simulink model "adc_zcu111"  (R2018a)
settings: Solver=VariableStepAuto  StartTime=0.0  StopTime=10.0  RelTol=1e-3
libraries: xbsIndex_r4 x50
settings Model: Creator=qwerty40  LastModifiedBy=qwerty40

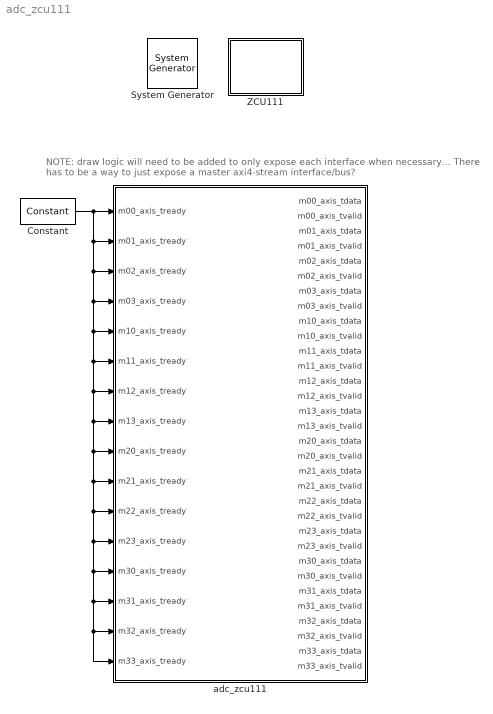
== system adc_zcu111 ==
  note: NOTE: draw logic will need to be added to only expose each interface when necessary...
      | There has to be a way to just expose a master axi4-stream interface/bus?
  " System Generator" : xbsIndex_r4/ System Generator  Tag=genX  xilinxfamily=zynquplusRFSOC  part=xczu28dr  speed=-2-e  package=ffvg1517  synthesis_tool=XST  clock_wrapper=Clock Enables  directory=/home/qwerty40/work_test/mlib_devel/xps_library/xps_models/ADCs/adc_zcu111/sysgen  proj_type=Vivado  Synth_file=Vivado Synthesis Defaults  Impl_file=Vivado Implementation Defaults  testbench=off  simulink_period=1  sysclk_period=10  dcm_input_clock_period=10  incr_netlist=off  trim_vbits=Everywhere in SubSystem  dbl_ovrd=According to Block Masks  core_generation=According to Block Masks  run_coregen=off  deprecated_control=off  eval_field=0  block_type=sysgen
  Constant : xbsIndex_r4/Constant  const=1.0  gui_display_data_type=Boolean  arith_type=Boolean  n_bits=16  bin_pt=14  preci_type=Single  exp_width=8  frac_width=24  explicit_period=off  period=1  equ=P=C  opselect=C  inp2=PCIN>>17  opr=+  inp1=P  carry=CIN  dbl_ovrd=off  block_type=constant
  ZCU111 : Subsystem  Tag=xps:xsg  mask(xsg core config){hw_sys=ZCU111:xczu28dr, clk_src=sys_clk, clk_rate=100, sample_period=1, synthesis_tool=XST}
      mask prompts: hw_sys "Hardware Platform"; clk_src "User IP Clock source"; clk_rate "User IP Clock Rate (MHz)"; sample_period "Sample Period"; synthesis_tool "Synthesis Tool:"
      mask help:
      | The XSG Core Config block is used to configure the System Generator design
      | for the casper_xps toolflow. Settings here are used to configure the
      | Xilinx System Generator block parameters automatically, and control toolflow
      | script  execution. It needs to be at the top level of all designs being compiled
      | with the casper_xps toolflow.
      mask init:
      | xps_xsg_zcu111_conf_mask;
      mask Help: eval('xlWeb([getenv(''MLIB_ROOT''), ''\doc\html\sys_xsg_core_config\sys_xsg_core_config.html''])')
      mask TypeOptions hw_sys: ZCU111:xczu28dr
      mask TypeOptions clk_src: sys_clk | adc_clk
      mask TypeOptions synthesis_tool: Leonardo Spectrum | Synplify | Synplify Pro | XST
      mask Display: fprintf(['ZCU111']);
  adc_zcu111 : Subsystem  Tag=xps:adc_zcu111  mask(adc_zcu111){tile_224_enable_pll=on, tile_224_sample_rate=4096, tile_224_clk_out=256.000, tile_224_ref_clk=512.000, tile_224_axi_stream_clk=0, tile_224_adc_0=on, tile_224_adc0_digital_output=I/Q, tile_224_adc0_dec_mode=2x, tile_224_adc0_sample_per_cycle=8, tile_224_adc0_req_axis_clk=0, tile_224_adc_1=on, tile_224_adc1_digital_output=I/Q, tile_224_adc1_dec_mode=2x, tile_224_adc1_sample_per_cycle=8, tile_224_adc1_req_axis_clk=0, tile_225_enable_pll=on, tile_225_sample_rate=4096, tile_225_clk_out=256.000, tile_225_ref_clk=512.000, tile_225_axi_stream_clk=0, tile_225_adc_0=on, tile_225_adc0_digital_output=I/Q, tile_225_adc0_dec_mode=2x, tile_225_adc0_sample_per_cycle=8, tile_225_adc0_req_axis_clk=0, tile_225_adc_1=on, tile_225_adc1_digital_output=I/Q, tile_225_adc1_dec_mode=2x, tile_225_adc1_sample_per_cycle=8, tile_225_adc1_req_axis_clk=0, tile_226_enable_pll=on, tile_226_sample_rate=4096, tile_226_clk_out=256.000, tile_226_ref_clk=512.000, tile_226_axi_stream_clk=0, tile_226_adc_0=on, tile_226_adc0_digital_output=I/Q, tile_226_adc0_dec_mode=2x, tile_226_adc0_sample_per_cycle=8, tile_226_adc0_req_axis_clk=0, tile_226_adc_1=on, tile_226_adc1_digital_output=I/Q, tile_226_adc1_dec_mode=2x, tile_226_adc1_sample_per_cycle=8, tile_226_adc1_req_axis_clk=0, tile_227_enable_pll=on, tile_227_sample_rate=4096, tile_227_clk_out=256.000, tile_227_ref_clk=512.000, tile_227_axi_stream_clk=0, tile_227_adc_0=on, tile_227_adc0_digital_output=I/Q, tile_227_adc0_dec_mode=2x, tile_227_adc0_sample_per_cycle=8, tile_227_adc0_req_axis_clk=0, tile_227_adc_1=on, tile_227_adc1_digital_output=I/Q, tile_227_adc1_dec_mode=2x, tile_227_adc1_sample_per_cycle=8, tile_227_adc1_req_axis_clk=0}
      mask prompts: tile_224_enable_pll "Enable PLL"; tile_224_sample_rate "Sampling Rate (MSPS)"; tile_224_clk_out "Clock Out (MHz)"; tile_224_ref_clk "Reference Clock (MHz)"; tile_224_axi_stream_clk "AXI4-Stream Clock (MHz)"; tile_224_adc_0 "Enable ADC"; tile_224_adc0_digital_output "Digital Output Data"; tile_224_adc0_dec_mode "Decimation Mode"; tile_224_adc0_sample_per_cycle "Samples per AXI4-Stream Cycle"; tile_224_adc_1 "Enable ADC"; tile_224_adc1_digital_output "Digital Output Data"; tile_224_adc1_dec_mode "Decimation Mode"; tile_224_adc1_sample_per_cycle "Samples per AXI4-Stream Cycle"; tile_225_enable_pll "Enable PLL"; tile_225_sample_rate "Sampling Rate (MSPS)"; tile_225_clk_out "Clock Out (MHz)"; tile_225_ref_clk "Reference Clock (MHz)"; tile_225_axi_stream_clk "AXI4-Stream Clock (MHz)"; tile_225_adc_0 "Enable ADC"; tile_225_adc0_digital_output "Digital Output Data"; tile_225_adc0_dec_mode "Decimation Mode"; tile_225_adc0_sample_per_cycle "Samples per AXI4-Stream Cycle"; tile_225_adc_1 "Enable ADC"; tile_225_adc1_digital_output "Digital Output Data"; tile_225_adc1_dec_mode "Decimation Mode"; tile_225_adc1_sample_per_cycle "Samples per AXI4-Stream Cycle"; tile_226_enable_pll "Enable PLL"; tile_226_sample_rate "Sampling Rate (MSPS)"; tile_226_clk_out "Clock Out (MHz)"; tile_226_ref_clk "Reference Clock (MHz)"; tile_226_axi_stream_clk "AXI4-Stream Clock (MHz)"; tile_226_adc_0 "Enable ADC"; tile_226_adc0_digital_output "Digital Output Data"; tile_226_adc0_dec_mode "Decimation Mode"; tile_226_adc0_sample_per_cycle "Samples per AXI4-Stream Cycle"; tile_226_adc_1 "Enable ADC"; tile_226_adc1_digital_output "Digital Output Data"; tile_226_adc1_dec_mode "Decimation Mode"; tile_226_adc1_sample_per_cycle "Samples per AXI4-Stream Cycle"; tile_227_enable_pll "Enable PLL"; tile_227_sample_rate "Sampling Rate (MSPS)"; tile_227_clk_out "Clock Out (MHz)"; tile_227_ref_clk "Reference Clock (MHz)"; tile_227_axi_stream_clk "AXI4-Stream Clock (MHz)"; tile_227_adc_0 "Enable ADC"; tile_227_adc0_digital_output "Digital Output Data"; tile_227_adc0_dec_mode "Decimation Mode"; tile_227_adc0_sample_per_cycle "Samples per AXI4-Stream Cycle"; tile_227_adc_1 "Enable ADC"; tile_227_adc1_digital_output "Digital Output Data"; tile_227_adc1_dec_mode "Decimation Mode"; tile_227_adc1_sample_per_cycle "Samples per AXI4-Stream Cycle"
      mask init:
      | %adc_zcu111_mask;
      mask Help: eval('xlWeb([getenv(''MLIB_ROOT''), ''\doc\html\adc_zcu111\adc_zcu111.html''])')
      mask TypeOptions tile_224_clk_out: 32.000 | 64.000 | 128.000 | 256.000
      mask TypeOptions tile_224_ref_clk: 103.261 | 104.136 | 105.026 | 105.931 | 106.852 | 107.790 | 108.743 | 109.714 | 110.703 | 111.709 | 112.734 | 113.778 | 114.841 | 115.925 | 117.029 | 118.154 | 119.301 | 120.471 | 121.663 | 122.880 | 124.121 | 125.388 | 126.680 | 128.000 | 129.347 | 130.723 | 132.129 | 133.565 | 135.033 | 136.533 | 138.067 | 139.636 | 141.241 | 142.884 | 144.565 | 146.286 | 148.048 | 149.854 | 151.704 | 153.600 | 155.544 | 157.539 | 159.584 | 161.684 | 163.840 | 166.054 | 168.329 | 170.667 | 173.070 | 175.543 | 178.087 | 180.706 | 183.403 | 186.182 | 189.046 | 192.000 | 195.048 | 198.194 | 201.443 | 204.800 | 208.271 | 211.862 | 215.579 | 219.429 | 223.418 | 227.556 | 231.849 | 236.308 | 240.941 | 245.760 | 250.776 | 256.000 | 261.447 | 267.130 | 273.067 | 279.273 | 285.767 | 292.571 | 299.707 | 307.200 | 315.077 | 323.368 | 332.108 | 341.333 | 351.086 | 361.412 | 372.364 | 384.000 | 396.387 | 409.600 | 423.724 | 438.857 | 455.111 | 472.615 | 491.520 | 512.000 | 534.261 | 558.546 | 585.143 | 614.400 | 646.737 | 682.667 | 722.824 | 768.000
      mask TypeOptions tile_224_adc0_digital_output: I/Q | Real
      mask TypeOptions tile_224_adc0_dec_mode: 1x | 2x | 4x | 8x
      mask TypeOptions tile_224_adc0_sample_per_cycle: 1 | 2 | 3 | 4 | 5 | 6 | 7 | 8
      mask TypeOptions tile_224_adc1_digital_output: I/Q | Real
      mask TypeOptions tile_224_adc1_dec_mode: 1x | 2x | 4x | 8x
      mask TypeOptions tile_224_adc1_sample_per_cycle: 1 | 2 | 3 | 4 | 5 | 6 | 7 | 8
      mask TypeOptions tile_225_clk_out: 32.000 | 64.000 | 128.000 | 256.000
      mask TypeOptions tile_225_ref_clk: 103.261 | 104.136 | 105.026 | 105.931 | 106.852 | 107.790 | 108.743 | 109.714 | 110.703 | 111.709 | 112.734 | 113.778 | 114.841 | 115.925 | 117.029 | 118.154 | 119.301 | 120.471 | 121.663 | 122.880 | 124.121 | 125.388 | 126.680 | 128.000 | 129.347 | 130.723 | 132.129 | 133.565 | 135.033 | 136.533 | 138.067 | 139.636 | 141.241 | 142.884 | 144.565 | 146.286 | 148.048 | 149.854 | 151.704 | 153.600 | 155.544 | 157.539 | 159.584 | 161.684 | 163.840 | 166.054 | 168.329 | 170.667 | 173.070 | 175.543 | 178.087 | 180.706 | 183.403 | 186.182 | 189.046 | 192.000 | 195.048 | 198.194 | 201.443 | 204.800 | 208.271 | 211.862 | 215.579 | 219.429 | 223.418 | 227.556 | 231.849 | 236.308 | 240.941 | 245.760 | 250.776 | 256.000 | 261.447 | 267.130 | 273.067 | 279.273 | 285.767 | 292.571 | 299.707 | 307.200 | 315.077 | 323.368 | 332.108 | 341.333 | 351.086 | 361.412 | 372.364 | 384.000 | 396.387 | 409.600 | 423.724 | 438.857 | 455.111 | 472.615 | 491.520 | 512.000 | 534.261 | 558.546 | 585.143 | 614.400 | 646.737 | 682.667 | 722.824 | 768.000
      mask TypeOptions tile_225_adc0_digital_output: I/Q | Real
      mask TypeOptions tile_225_adc0_dec_mode: 1x | 2x | 4x | 8x
      mask TypeOptions tile_225_adc0_sample_per_cycle: 1 | 2 | 3 | 4 | 5 | 6 | 7 | 8
      mask TypeOptions tile_225_adc1_digital_output: I/Q | Real
      mask TypeOptions tile_225_adc1_dec_mode: 1x | 2x | 4x | 8x
      mask TypeOptions tile_225_adc1_sample_per_cycle: 1 | 2 | 3 | 4 | 5 | 6 | 7 | 8
      mask TypeOptions tile_226_clk_out: 32.000 | 64.000 | 128.000 | 256.000
      mask TypeOptions tile_226_ref_clk: 103.261 | 104.136 | 105.026 | 105.931 | 106.852 | 107.790 | 108.743 | 109.714 | 110.703 | 111.709 | 112.734 | 113.778 | 114.841 | 115.925 | 117.029 | 118.154 | 119.301 | 120.471 | 121.663 | 122.880 | 124.121 | 125.388 | 126.680 | 128.000 | 129.347 | 130.723 | 132.129 | 133.565 | 135.033 | 136.533 | 138.067 | 139.636 | 141.241 | 142.884 | 144.565 | 146.286 | 148.048 | 149.854 | 151.704 | 153.600 | 155.544 | 157.539 | 159.584 | 161.684 | 163.840 | 166.054 | 168.329 | 170.667 | 173.070 | 175.543 | 178.087 | 180.706 | 183.403 | 186.182 | 189.046 | 192.000 | 195.048 | 198.194 | 201.443 | 204.800 | 208.271 | 211.862 | 215.579 | 219.429 | 223.418 | 227.556 | 231.849 | 236.308 | 240.941 | 245.760 | 250.776 | 256.000 | 261.447 | 267.130 | 273.067 | 279.273 | 285.767 | 292.571 | 299.707 | 307.200 | 315.077 | 323.368 | 332.108 | 341.333 | 351.086 | 361.412 | 372.364 | 384.000 | 396.387 | 409.600 | 423.724 | 438.857 | 455.111 | 472.615 | 491.520 | 512.000 | 534.261 | 558.546 | 585.143 | 614.400 | 646.737 | 682.667 | 722.824 | 768.000
      mask TypeOptions tile_226_adc0_digital_output: I/Q | Real
      mask TypeOptions tile_226_adc0_dec_mode: 1x | 2x | 4x | 8x
      mask TypeOptions tile_226_adc0_sample_per_cycle: 1 | 2 | 3 | 4 | 5 | 6 | 7 | 8
      mask TypeOptions tile_226_adc1_digital_output: I/Q | Real
      mask TypeOptions tile_226_adc1_dec_mode: 1x | 2x | 4x | 8x
      mask TypeOptions tile_226_adc1_sample_per_cycle: 1 | 2 | 3 | 4 | 5 | 6 | 7 | 8
      mask TypeOptions tile_227_clk_out: 32.000 | 64.000 | 128.000 | 256.000
      mask TypeOptions tile_227_ref_clk: 103.261 | 104.136 | 105.026 | 105.931 | 106.852 | 107.790 | 108.743 | 109.714 | 110.703 | 111.709 | 112.734 | 113.778 | 114.841 | 115.925 | 117.029 | 118.154 | 119.301 | 120.471 | 121.663 | 122.880 | 124.121 | 125.388 | 126.680 | 128.000 | 129.347 | 130.723 | 132.129 | 133.565 | 135.033 | 136.533 | 138.067 | 139.636 | 141.241 | 142.884 | 144.565 | 146.286 | 148.048 | 149.854 | 151.704 | 153.600 | 155.544 | 157.539 | 159.584 | 161.684 | 163.840 | 166.054 | 168.329 | 170.667 | 173.070 | 175.543 | 178.087 | 180.706 | 183.403 | 186.182 | 189.046 | 192.000 | 195.048 | 198.194 | 201.443 | 204.800 | 208.271 | 211.862 | 215.579 | 219.429 | 223.418 | 227.556 | 231.849 | 236.308 | 240.941 | 245.760 | 250.776 | 256.000 | 261.447 | 267.130 | 273.067 | 279.273 | 285.767 | 292.571 | 299.707 | 307.200 | 315.077 | 323.368 | 332.108 | 341.333 | 351.086 | 361.412 | 372.364 | 384.000 | 396.387 | 409.600 | 423.724 | 438.857 | 455.111 | 472.615 | 491.520 | 512.000 | 534.261 | 558.546 | 585.143 | 614.400 | 646.737 | 682.667 | 722.824 | 768.000
      mask TypeOptions tile_227_adc0_digital_output: I/Q | Real
      mask TypeOptions tile_227_adc0_dec_mode: 1x | 2x | 4x | 8x
      mask TypeOptions tile_227_adc0_sample_per_cycle: 1 | 2 | 3 | 4 | 5 | 6 | 7 | 8
      mask TypeOptions tile_227_adc1_digital_output: I/Q | Real
      mask TypeOptions tile_227_adc1_dec_mode: 1x | 2x | 4x | 8x
      mask TypeOptions tile_227_adc1_sample_per_cycle: 1 | 2 | 3 | 4 | 5 | 6 | 7 | 8
      mask DialogControl adc_tile_224 Prompt: ADC Tile 224
      mask DialogControl pll_clocking_config_224 Prompt: PLL and Clocking Configuration
      mask DialogControl tile_224_adc0 Prompt: ADC 0
      mask DialogControl tile_224_adc0_data_settings Prompt: Data Settings
      mask DialogControl tile_224_adc0_req_axis_clk_label Prompt: Required AXI4-Stream clock:
      mask DialogControl tile_224_adc1 Prompt: ADC 1
      mask DialogControl tile_224_adc1_data_settings Prompt: Data Settings
      mask DialogControl tile_224_adc1_req_axis_clk_label Prompt: Required AXI4-Stream clock:
      mask DialogControl adc_tile_225 Prompt: ADC Tile 225
      mask DialogControl pll_clocking_config_225 Prompt: PLL and Clocking Configuration
      mask DialogControl tile_225_adc0 Prompt: ADC 0
      mask DialogControl tile_225_adc0_data_settings Prompt: Data Settings
      mask DialogControl tile_225_adc0_req_axis_clk_label Prompt: Required AXI4-Stream clock:
      mask DialogControl tile_225_adc1 Prompt: ADC 1
      mask DialogControl tile_225_adc1_data_settings Prompt: Data Settings
      mask DialogControl tile_225_adc1_req_axis_clk_label Prompt: Required AXI4-Stream clock:
      mask DialogControl adc_tile_226 Prompt: ADC Tile 226
      mask DialogControl pll_clocking_config_226 Prompt: PLL and Clocking Configuration
      mask DialogControl tile_226_adc0 Prompt: ADC 0
      mask DialogControl tile_226_adc0_data_settings Prompt: Data Settings
      mask DialogControl tile_226_adc0_req_axis_clk_label Prompt: Required AXI4-Stream clock:
      mask DialogControl tile_226_adc1 Prompt: ADC 1
      mask DialogControl tile_226_adc1_data_settings Prompt: Data Settings
      mask DialogControl tile_226_adc1_req_axis_clk_label Prompt: Required AXI4-Stream clock:
      mask DialogControl adc_tile_227 Prompt: ADC Tile 227
      mask DialogControl pll_clocking_config_227 Prompt: PLL and Clocking Configuration
      mask DialogControl tile_227_adc0 Prompt: ADC 0
      mask DialogControl tile_227_adc0_data_settings Prompt: Data Settings
      mask DialogControl tile_227_adc0_req_axis_clk_label Prompt: Required AXI4-Stream clock:
      mask DialogControl tile_227_adc1 Prompt: ADC 1
      mask DialogControl tile_227_adc1_data_settings Prompt: Data Settings
      mask DialogControl tile_227_adc1_req_axis_clk_label Prompt: Required AXI4-Stream clock:
  wires:
  Constant/1 -> adc_zcu111/4(m03_axis_tready), adc_zcu111/5(m10_axis_tready), adc_zcu111/6(m11_axis_tready), adc_zcu111/7(m12_axis_tready), adc_zcu111/8(m13_axis_tready), adc_zcu111/9(m20_axis_tready), adc_zcu111/10(m21_axis_tready), adc_zcu111/11(m22_axis_tready), adc_zcu111/13(m30_axis_tready), adc_zcu111/14(m31_axis_tready), adc_zcu111/15(m32_axis_tready), adc_zcu111/16(m33_axis_tready), adc_zcu111/12(m23_axis_tready), adc_zcu111/3(m02_axis_tready), adc_zcu111/2(m01_axis_tready), adc_zcu111/1(m00_axis_tready)

== system adc_zcu111/ZCU111 ==

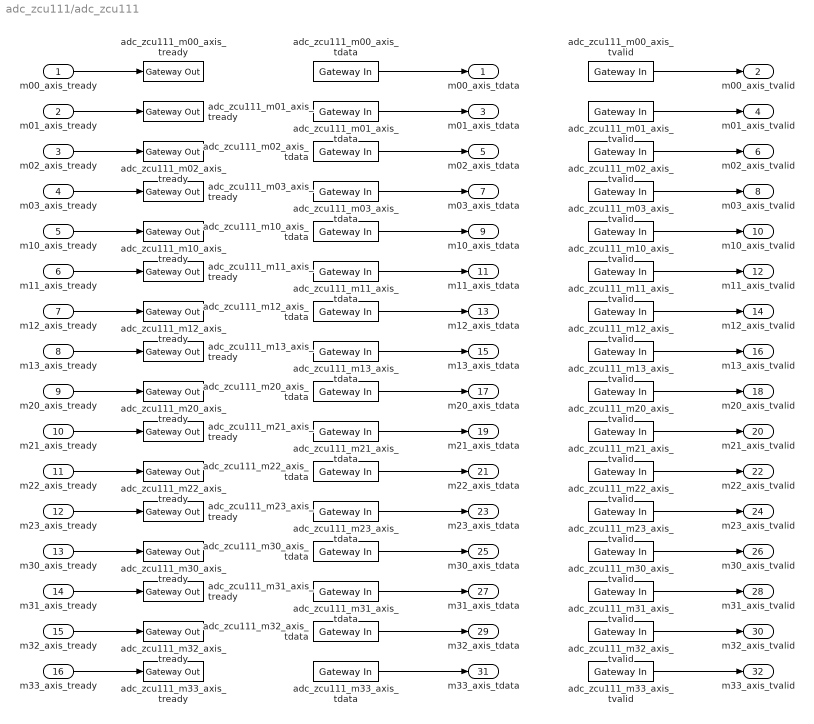
== system adc_zcu111/adc_zcu111 ==
  m00_axis_tready : Inport  OutDataTypeStr=boolean
  m01_axis_tready : Inport  Port=2  OutDataTypeStr=boolean
  m02_axis_tready : Inport  Port=3  OutDataTypeStr=boolean
  m03_axis_tready : Inport  Port=4  OutDataTypeStr=boolean
  m10_axis_tready : Inport  Port=5  OutDataTypeStr=boolean
  m11_axis_tready : Inport  Port=6  OutDataTypeStr=boolean
  m12_axis_tready : Inport  Port=7  OutDataTypeStr=boolean
  m13_axis_tready : Inport  Port=8  OutDataTypeStr=boolean
  m20_axis_tready : Inport  Port=9  OutDataTypeStr=boolean
  m21_axis_tready : Inport  Port=10  OutDataTypeStr=boolean
  m22_axis_tready : Inport  Port=11  OutDataTypeStr=boolean
  m23_axis_tready : Inport  Port=12  OutDataTypeStr=boolean
  m30_axis_tready : Inport  Port=13  OutDataTypeStr=boolean
  m31_axis_tready : Inport  Port=14  OutDataTypeStr=boolean
  m32_axis_tready : Inport  Port=15  OutDataTypeStr=boolean
  m33_axis_tready : Inport  Port=16  OutDataTypeStr=boolean
  adc_zcu111_m00_axis_tdata : xbsIndex_r4/Gateway In  gui_display_data_type=Fixed-point  arith_type="Signed  (2's comp)"  n_bits=128  bin_pt=126  preci_type=Double  exp_width=8  frac_width=24  rows=1  columns=1  quantization="Round  (unbiased: +/- Inf)"  overflow=Saturate  period=1  UseAsADC=off  ADCChannel='1'  interface=None  automatic_assignment=on  address_offset=hex2dec('00')  intf_name=''  intf_description=''  default_value=0  timing_constraint=None  locs_specified=off  LOCs={}  io_standard={}  inherit_from_input=off  hdl_port=on  dbl_ovrd=off  block_type=gatewayin
  adc_zcu111_m00_axis_tready : xbsIndex_r4/Gateway Out  inherit_from_input=on  hdl_port=on  rows=1  columns=1  UseAsDAC=off  DACChannel='1'  interface=None  automatic_assignment=on  address_offset=hex2dec('00')  intf_name=''  intf_description=''  timing_constraint=None  locs_specified=off  LOCs={}  io_standard={}  block_type=gatewayout
  adc_zcu111_m00_axis_tvalid : xbsIndex_r4/Gateway In  gui_display_data_type=Boolean  arith_type=Boolean  n_bits=128  bin_pt=126  preci_type=Double  exp_width=8  frac_width=24  rows=1  columns=1  quantization="Round  (unbiased: +/- Inf)"  overflow=Saturate  period=1  UseAsADC=off  ADCChannel='1'  interface=None  automatic_assignment=on  address_offset=hex2dec('00')  intf_name=''  intf_description=''  default_value=0  timing_constraint=None  locs_specified=off  LOCs={}  io_standard={}  inherit_from_input=off  hdl_port=on  dbl_ovrd=off  block_type=gatewayin
  adc_zcu111_m01_axis_tdata : xbsIndex_r4/Gateway In  gui_display_data_type=Fixed-point  arith_type="Signed  (2's comp)"  n_bits=128  bin_pt=126  preci_type=Double  exp_width=8  frac_width=24  rows=1  columns=1  quantization="Round  (unbiased: +/- Inf)"  overflow=Saturate  period=1  UseAsADC=off  ADCChannel='1'  interface=None  automatic_assignment=on  address_offset=hex2dec('00')  intf_name=''  intf_description=''  default_value=0  timing_constraint=None  locs_specified=off  LOCs={}  io_standard={}  inherit_from_input=off  hdl_port=on  dbl_ovrd=off  block_type=gatewayin
  adc_zcu111_m01_axis_tready : xbsIndex_r4/Gateway Out  inherit_from_input=on  hdl_port=on  rows=1  columns=1  UseAsDAC=off  DACChannel='1'  interface=None  automatic_assignment=on  address_offset=hex2dec('00')  intf_name=''  intf_description=''  timing_constraint=None  locs_specified=off  LOCs={}  io_standard={}  block_type=gatewayout
  adc_zcu111_m01_axis_tvalid : xbsIndex_r4/Gateway In  gui_display_data_type=Boolean  arith_type=Boolean  n_bits=128  bin_pt=126  preci_type=Double  exp_width=8  frac_width=24  rows=1  columns=1  quantization="Round  (unbiased: +/- Inf)"  overflow=Saturate  period=1  UseAsADC=off  ADCChannel='1'  interface=None  automatic_assignment=on  address_offset=hex2dec('00')  intf_name=''  intf_description=''  default_value=0  timing_constraint=None  locs_specified=off  LOCs={}  io_standard={}  inherit_from_input=off  hdl_port=on  dbl_ovrd=off  block_type=gatewayin
  adc_zcu111_m02_axis_tdata : xbsIndex_r4/Gateway In  gui_display_data_type=Fixed-point  arith_type="Signed  (2's comp)"  n_bits=128  bin_pt=126  preci_type=Double  exp_width=8  frac_width=24  rows=1  columns=1  quantization="Round  (unbiased: +/- Inf)"  overflow=Saturate  period=1  UseAsADC=off  ADCChannel='1'  interface=None  automatic_assignment=on  address_offset=hex2dec('00')  intf_name=''  intf_description=''  default_value=0  timing_constraint=None  locs_specified=off  LOCs={}  io_standard={}  inherit_from_input=off  hdl_port=on  dbl_ovrd=off  block_type=gatewayin
  adc_zcu111_m02_axis_tready : xbsIndex_r4/Gateway Out  inherit_from_input=on  hdl_port=on  rows=1  columns=1  UseAsDAC=off  DACChannel='1'  interface=None  automatic_assignment=on  address_offset=hex2dec('00')  intf_name=''  intf_description=''  timing_constraint=None  locs_specified=off  LOCs={}  io_standard={}  block_type=gatewayout
  adc_zcu111_m02_axis_tvalid : xbsIndex_r4/Gateway In  gui_display_data_type=Boolean  arith_type=Boolean  n_bits=128  bin_pt=126  preci_type=Double  exp_width=8  frac_width=24  rows=1  columns=1  quantization="Round  (unbiased: +/- Inf)"  overflow=Saturate  period=1  UseAsADC=off  ADCChannel='1'  interface=None  automatic_assignment=on  address_offset=hex2dec('00')  intf_name=''  intf_description=''  default_value=0  timing_constraint=None  locs_specified=off  LOCs={}  io_standard={}  inherit_from_input=off  hdl_port=on  dbl_ovrd=off  block_type=gatewayin
  adc_zcu111_m03_axis_tdata : xbsIndex_r4/Gateway In  gui_display_data_type=Fixed-point  arith_type="Signed  (2's comp)"  n_bits=128  bin_pt=126  preci_type=Double  exp_width=8  frac_width=24  rows=1  columns=1  quantization="Round  (unbiased: +/- Inf)"  overflow=Saturate  period=1  UseAsADC=off  ADCChannel='1'  interface=None  automatic_assignment=on  address_offset=hex2dec('00')  intf_name=''  intf_description=''  default_value=0  timing_constraint=None  locs_specified=off  LOCs={}  io_standard={}  inherit_from_input=off  hdl_port=on  dbl_ovrd=off  block_type=gatewayin
  adc_zcu111_m03_axis_tready : xbsIndex_r4/Gateway Out  inherit_from_input=on  hdl_port=on  rows=1  columns=1  UseAsDAC=off  DACChannel='1'  interface=None  automatic_assignment=on  address_offset=hex2dec('00')  intf_name=''  intf_description=''  timing_constraint=None  locs_specified=off  LOCs={}  io_standard={}  block_type=gatewayout
  adc_zcu111_m03_axis_tvalid : xbsIndex_r4/Gateway In  gui_display_data_type=Boolean  arith_type=Boolean  n_bits=128  bin_pt=126  preci_type=Double  exp_width=8  frac_width=24  rows=1  columns=1  quantization="Round  (unbiased: +/- Inf)"  overflow=Saturate  period=1  UseAsADC=off  ADCChannel='1'  interface=None  automatic_assignment=on  address_offset=hex2dec('00')  intf_name=''  intf_description=''  default_value=0  timing_constraint=None  locs_specified=off  LOCs={}  io_standard={}  inherit_from_input=off  hdl_port=on  dbl_ovrd=off  block_type=gatewayin
  adc_zcu111_m10_axis_tdata : xbsIndex_r4/Gateway In  gui_display_data_type=Fixed-point  arith_type="Signed  (2's comp)"  n_bits=128  bin_pt=126  preci_type=Double  exp_width=8  frac_width=24  rows=1  columns=1  quantization="Round  (unbiased: +/- Inf)"  overflow=Saturate  period=1  UseAsADC=off  ADCChannel='1'  interface=None  automatic_assignment=on  address_offset=hex2dec('00')  intf_name=''  intf_description=''  default_value=0  timing_constraint=None  locs_specified=off  LOCs={}  io_standard={}  inherit_from_input=off  hdl_port=on  dbl_ovrd=off  block_type=gatewayin
  adc_zcu111_m10_axis_tready : xbsIndex_r4/Gateway Out  inherit_from_input=on  hdl_port=on  rows=1  columns=1  UseAsDAC=off  DACChannel='1'  interface=None  automatic_assignment=on  address_offset=hex2dec('00')  intf_name=''  intf_description=''  timing_constraint=None  locs_specified=off  LOCs={}  io_standard={}  block_type=gatewayout
  adc_zcu111_m10_axis_tvalid : xbsIndex_r4/Gateway In  gui_display_data_type=Boolean  arith_type=Boolean  n_bits=128  bin_pt=126  preci_type=Double  exp_width=8  frac_width=24  rows=1  columns=1  quantization="Round  (unbiased: +/- Inf)"  overflow=Saturate  period=1  UseAsADC=off  ADCChannel='1'  interface=None  automatic_assignment=on  address_offset=hex2dec('00')  intf_name=''  intf_description=''  default_value=0  timing_constraint=None  locs_specified=off  LOCs={}  io_standard={}  inherit_from_input=off  hdl_port=on  dbl_ovrd=off  block_type=gatewayin
  adc_zcu111_m11_axis_tdata : xbsIndex_r4/Gateway In  gui_display_data_type=Fixed-point  arith_type="Signed  (2's comp)"  n_bits=128  bin_pt=126  preci_type=Double  exp_width=8  frac_width=24  rows=1  columns=1  quantization="Round  (unbiased: +/- Inf)"  overflow=Saturate  period=1  UseAsADC=off  ADCChannel='1'  interface=None  automatic_assignment=on  address_offset=hex2dec('00')  intf_name=''  intf_description=''  default_value=0  timing_constraint=None  locs_specified=off  LOCs={}  io_standard={}  inherit_from_input=off  hdl_port=on  dbl_ovrd=off  block_type=gatewayin
  adc_zcu111_m11_axis_tready : xbsIndex_r4/Gateway Out  inherit_from_input=on  hdl_port=on  rows=1  columns=1  UseAsDAC=off  DACChannel='1'  interface=None  automatic_assignment=on  address_offset=hex2dec('00')  intf_name=''  intf_description=''  timing_constraint=None  locs_specified=off  LOCs={}  io_standard={}  block_type=gatewayout
  adc_zcu111_m11_axis_tvalid : xbsIndex_r4/Gateway In  gui_display_data_type=Boolean  arith_type=Boolean  n_bits=128  bin_pt=126  preci_type=Double  exp_width=8  frac_width=24  rows=1  columns=1  quantization="Round  (unbiased: +/- Inf)"  overflow=Saturate  period=1  UseAsADC=off  ADCChannel='1'  interface=None  automatic_assignment=on  address_offset=hex2dec('00')  intf_name=''  intf_description=''  default_value=0  timing_constraint=None  locs_specified=off  LOCs={}  io_standard={}  inherit_from_input=off  hdl_port=on  dbl_ovrd=off  block_type=gatewayin
  adc_zcu111_m12_axis_tdata : xbsIndex_r4/Gateway In  gui_display_data_type=Fixed-point  arith_type="Signed  (2's comp)"  n_bits=128  bin_pt=126  preci_type=Double  exp_width=8  frac_width=24  rows=1  columns=1  quantization="Round  (unbiased: +/- Inf)"  overflow=Saturate  period=1  UseAsADC=off  ADCChannel='1'  interface=None  automatic_assignment=on  address_offset=hex2dec('00')  intf_name=''  intf_description=''  default_value=0  timing_constraint=None  locs_specified=off  LOCs={}  io_standard={}  inherit_from_input=off  hdl_port=on  dbl_ovrd=off  block_type=gatewayin
  adc_zcu111_m12_axis_tready : xbsIndex_r4/Gateway Out  inherit_from_input=on  hdl_port=on  rows=1  columns=1  UseAsDAC=off  DACChannel='1'  interface=None  automatic_assignment=on  address_offset=hex2dec('00')  intf_name=''  intf_description=''  timing_constraint=None  locs_specified=off  LOCs={}  io_standard={}  block_type=gatewayout
  adc_zcu111_m12_axis_tvalid : xbsIndex_r4/Gateway In  gui_display_data_type=Boolean  arith_type=Boolean  n_bits=128  bin_pt=126  preci_type=Double  exp_width=8  frac_width=24  rows=1  columns=1  quantization="Round  (unbiased: +/- Inf)"  overflow=Saturate  period=1  UseAsADC=off  ADCChannel='1'  interface=None  automatic_assignment=on  address_offset=hex2dec('00')  intf_name=''  intf_description=''  default_value=0  timing_constraint=None  locs_specified=off  LOCs={}  io_standard={}  inherit_from_input=off  hdl_port=on  dbl_ovrd=off  block_type=gatewayin
  adc_zcu111_m13_axis_tdata : xbsIndex_r4/Gateway In  gui_display_data_type=Fixed-point  arith_type="Signed  (2's comp)"  n_bits=128  bin_pt=126  preci_type=Double  exp_width=8  frac_width=24  rows=1  columns=1  quantization="Round  (unbiased: +/- Inf)"  overflow=Saturate  period=1  UseAsADC=off  ADCChannel='1'  interface=None  automatic_assignment=on  address_offset=hex2dec('00')  intf_name=''  intf_description=''  default_value=0  timing_constraint=None  locs_specified=off  LOCs={}  io_standard={}  inherit_from_input=off  hdl_port=on  dbl_ovrd=off  block_type=gatewayin
  adc_zcu111_m13_axis_tready : xbsIndex_r4/Gateway Out  inherit_from_input=on  hdl_port=on  rows=1  columns=1  UseAsDAC=off  DACChannel='1'  interface=None  automatic_assignment=on  address_offset=hex2dec('00')  intf_name=''  intf_description=''  timing_constraint=None  locs_specified=off  LOCs={}  io_standard={}  block_type=gatewayout
  adc_zcu111_m13_axis_tvalid : xbsIndex_r4/Gateway In  gui_display_data_type=Boolean  arith_type=Boolean  n_bits=128  bin_pt=126  preci_type=Double  exp_width=8  frac_width=24  rows=1  columns=1  quantization="Round  (unbiased: +/- Inf)"  overflow=Saturate  period=1  UseAsADC=off  ADCChannel='1'  interface=None  automatic_assignment=on  address_offset=hex2dec('00')  intf_name=''  intf_description=''  default_value=0  timing_constraint=None  locs_specified=off  LOCs={}  io_standard={}  inherit_from_input=off  hdl_port=on  dbl_ovrd=off  block_type=gatewayin
  adc_zcu111_m20_axis_tdata : xbsIndex_r4/Gateway In  gui_display_data_type=Fixed-point  arith_type="Signed  (2's comp)"  n_bits=128  bin_pt=126  preci_type=Double  exp_width=8  frac_width=24  rows=1  columns=1  quantization="Round  (unbiased: +/- Inf)"  overflow=Saturate  period=1  UseAsADC=off  ADCChannel='1'  interface=None  automatic_assignment=on  address_offset=hex2dec('00')  intf_name=''  intf_description=''  default_value=0  timing_constraint=None  locs_specified=off  LOCs={}  io_standard={}  inherit_from_input=off  hdl_port=on  dbl_ovrd=off  block_type=gatewayin
  adc_zcu111_m20_axis_tready : xbsIndex_r4/Gateway Out  inherit_from_input=on  hdl_port=on  rows=1  columns=1  UseAsDAC=off  DACChannel='1'  interface=None  automatic_assignment=on  address_offset=hex2dec('00')  intf_name=''  intf_description=''  timing_constraint=None  locs_specified=off  LOCs={}  io_standard={}  block_type=gatewayout
  adc_zcu111_m20_axis_tvalid : xbsIndex_r4/Gateway In  gui_display_data_type=Boolean  arith_type=Boolean  n_bits=128  bin_pt=126  preci_type=Double  exp_width=8  frac_width=24  rows=1  columns=1  quantization="Round  (unbiased: +/- Inf)"  overflow=Saturate  period=1  UseAsADC=off  ADCChannel='1'  interface=None  automatic_assignment=on  address_offset=hex2dec('00')  intf_name=''  intf_description=''  default_value=0  timing_constraint=None  locs_specified=off  LOCs={}  io_standard={}  inherit_from_input=off  hdl_port=on  dbl_ovrd=off  block_type=gatewayin
  adc_zcu111_m21_axis_tdata : xbsIndex_r4/Gateway In  gui_display_data_type=Fixed-point  arith_type="Signed  (2's comp)"  n_bits=128  bin_pt=126  preci_type=Double  exp_width=8  frac_width=24  rows=1  columns=1  quantization="Round  (unbiased: +/- Inf)"  overflow=Saturate  period=1  UseAsADC=off  ADCChannel='1'  interface=None  automatic_assignment=on  address_offset=hex2dec('00')  intf_name=''  intf_description=''  default_value=0  timing_constraint=None  locs_specified=off  LOCs={}  io_standard={}  inherit_from_input=off  hdl_port=on  dbl_ovrd=off  block_type=gatewayin
  adc_zcu111_m21_axis_tready : xbsIndex_r4/Gateway Out  inherit_from_input=on  hdl_port=on  rows=1  columns=1  UseAsDAC=off  DACChannel='1'  interface=None  automatic_assignment=on  address_offset=hex2dec('00')  intf_name=''  intf_description=''  timing_constraint=None  locs_specified=off  LOCs={}  io_standard={}  block_type=gatewayout
  adc_zcu111_m21_axis_tvalid : xbsIndex_r4/Gateway In  gui_display_data_type=Boolean  arith_type=Boolean  n_bits=128  bin_pt=126  preci_type=Double  exp_width=8  frac_width=24  rows=1  columns=1  quantization="Round  (unbiased: +/- Inf)"  overflow=Saturate  period=1  UseAsADC=off  ADCChannel='1'  interface=None  automatic_assignment=on  address_offset=hex2dec('00')  intf_name=''  intf_description=''  default_value=0  timing_constraint=None  locs_specified=off  LOCs={}  io_standard={}  inherit_from_input=off  hdl_port=on  dbl_ovrd=off  block_type=gatewayin
  adc_zcu111_m22_axis_tdata : xbsIndex_r4/Gateway In  gui_display_data_type=Fixed-point  arith_type="Signed  (2's comp)"  n_bits=128  bin_pt=126  preci_type=Double  exp_width=8  frac_width=24  rows=1  columns=1  quantization="Round  (unbiased: +/- Inf)"  overflow=Saturate  period=1  UseAsADC=off  ADCChannel='1'  interface=None  automatic_assignment=on  address_offset=hex2dec('00')  intf_name=''  intf_description=''  default_value=0  timing_constraint=None  locs_specified=off  LOCs={}  io_standard={}  inherit_from_input=off  hdl_port=on  dbl_ovrd=off  block_type=gatewayin
  adc_zcu111_m22_axis_tready : xbsIndex_r4/Gateway Out  inherit_from_input=on  hdl_port=on  rows=1  columns=1  UseAsDAC=off  DACChannel='1'  interface=None  automatic_assignment=on  address_offset=hex2dec('00')  intf_name=''  intf_description=''  timing_constraint=None  locs_specified=off  LOCs={}  io_standard={}  block_type=gatewayout
  adc_zcu111_m22_axis_tvalid : xbsIndex_r4/Gateway In  gui_display_data_type=Boolean  arith_type=Boolean  n_bits=128  bin_pt=126  preci_type=Double  exp_width=8  frac_width=24  rows=1  columns=1  quantization="Round  (unbiased: +/- Inf)"  overflow=Saturate  period=1  UseAsADC=off  ADCChannel='1'  interface=None  automatic_assignment=on  address_offset=hex2dec('00')  intf_name=''  intf_description=''  default_value=0  timing_constraint=None  locs_specified=off  LOCs={}  io_standard={}  inherit_from_input=off  hdl_port=on  dbl_ovrd=off  block_type=gatewayin
  adc_zcu111_m23_axis_tdata : xbsIndex_r4/Gateway In  gui_display_data_type=Fixed-point  arith_type="Signed  (2's comp)"  n_bits=128  bin_pt=126  preci_type=Double  exp_width=8  frac_width=24  rows=1  columns=1  quantization="Round  (unbiased: +/- Inf)"  overflow=Saturate  period=1  UseAsADC=off  ADCChannel='1'  interface=None  automatic_assignment=on  address_offset=hex2dec('00')  intf_name=''  intf_description=''  default_value=0  timing_constraint=None  locs_specified=off  LOCs={}  io_standard={}  inherit_from_input=off  hdl_port=on  dbl_ovrd=off  block_type=gatewayin
  adc_zcu111_m23_axis_tready : xbsIndex_r4/Gateway Out  inherit_from_input=on  hdl_port=on  rows=1  columns=1  UseAsDAC=off  DACChannel='1'  interface=None  automatic_assignment=on  address_offset=hex2dec('00')  intf_name=''  intf_description=''  timing_constraint=None  locs_specified=off  LOCs={}  io_standard={}  block_type=gatewayout
  adc_zcu111_m23_axis_tvalid : xbsIndex_r4/Gateway In  gui_display_data_type=Boolean  arith_type=Boolean  n_bits=128  bin_pt=126  preci_type=Double  exp_width=8  frac_width=24  rows=1  columns=1  quantization="Round  (unbiased: +/- Inf)"  overflow=Saturate  period=1  UseAsADC=off  ADCChannel='1'  interface=None  automatic_assignment=on  address_offset=hex2dec('00')  intf_name=''  intf_description=''  default_value=0  timing_constraint=None  locs_specified=off  LOCs={}  io_standard={}  inherit_from_input=off  hdl_port=on  dbl_ovrd=off  block_type=gatewayin
  adc_zcu111_m30_axis_tdata : xbsIndex_r4/Gateway In  gui_display_data_type=Fixed-point  arith_type="Signed  (2's comp)"  n_bits=128  bin_pt=126  preci_type=Double  exp_width=8  frac_width=24  rows=1  columns=1  quantization="Round  (unbiased: +/- Inf)"  overflow=Saturate  period=1  UseAsADC=off  ADCChannel='1'  interface=None  automatic_assignment=on  address_offset=hex2dec('00')  intf_name=''  intf_description=''  default_value=0  timing_constraint=None  locs_specified=off  LOCs={}  io_standard={}  inherit_from_input=off  hdl_port=on  dbl_ovrd=off  block_type=gatewayin
  adc_zcu111_m30_axis_tready : xbsIndex_r4/Gateway Out  inherit_from_input=on  hdl_port=on  rows=1  columns=1  UseAsDAC=off  DACChannel='1'  interface=None  automatic_assignment=on  address_offset=hex2dec('00')  intf_name=''  intf_description=''  timing_constraint=None  locs_specified=off  LOCs={}  io_standard={}  block_type=gatewayout
  adc_zcu111_m30_axis_tvalid : xbsIndex_r4/Gateway In  gui_display_data_type=Boolean  arith_type=Boolean  n_bits=128  bin_pt=126  preci_type=Double  exp_width=8  frac_width=24  rows=1  columns=1  quantization="Round  (unbiased: +/- Inf)"  overflow=Saturate  period=1  UseAsADC=off  ADCChannel='1'  interface=None  automatic_assignment=on  address_offset=hex2dec('00')  intf_name=''  intf_description=''  default_value=0  timing_constraint=None  locs_specified=off  LOCs={}  io_standard={}  inherit_from_input=off  hdl_port=on  dbl_ovrd=off  block_type=gatewayin
  adc_zcu111_m31_axis_tdata : xbsIndex_r4/Gateway In  gui_display_data_type=Fixed-point  arith_type="Signed  (2's comp)"  n_bits=128  bin_pt=126  preci_type=Double  exp_width=8  frac_width=24  rows=1  columns=1  quantization="Round  (unbiased: +/- Inf)"  overflow=Saturate  period=1  UseAsADC=off  ADCChannel='1'  interface=None  automatic_assignment=on  address_offset=hex2dec('00')  intf_name=''  intf_description=''  default_value=0  timing_constraint=None  locs_specified=off  LOCs={}  io_standard={}  inherit_from_input=off  hdl_port=on  dbl_ovrd=off  block_type=gatewayin
  adc_zcu111_m31_axis_tready : xbsIndex_r4/Gateway Out  inherit_from_input=on  hdl_port=on  rows=1  columns=1  UseAsDAC=off  DACChannel='1'  interface=None  automatic_assignment=on  address_offset=hex2dec('00')  intf_name=''  intf_description=''  timing_constraint=None  locs_specified=off  LOCs={}  io_standard={}  block_type=gatewayout
  adc_zcu111_m31_axis_tvalid : xbsIndex_r4/Gateway In  gui_display_data_type=Boolean  arith_type=Boolean  n_bits=128  bin_pt=126  preci_type=Double  exp_width=8  frac_width=24  rows=1  columns=1  quantization="Round  (unbiased: +/- Inf)"  overflow=Saturate  period=1  UseAsADC=off  ADCChannel='1'  interface=None  automatic_assignment=on  address_offset=hex2dec('00')  intf_name=''  intf_description=''  default_value=0  timing_constraint=None  locs_specified=off  LOCs={}  io_standard={}  inherit_from_input=off  hdl_port=on  dbl_ovrd=off  block_type=gatewayin
  adc_zcu111_m32_axis_tdata : xbsIndex_r4/Gateway In  gui_display_data_type=Fixed-point  arith_type="Signed  (2's comp)"  n_bits=128  bin_pt=126  preci_type=Double  exp_width=8  frac_width=24  rows=1  columns=1  quantization="Round  (unbiased: +/- Inf)"  overflow=Saturate  period=1  UseAsADC=off  ADCChannel='1'  interface=None  automatic_assignment=on  address_offset=hex2dec('00')  intf_name=''  intf_description=''  default_value=0  timing_constraint=None  locs_specified=off  LOCs={}  io_standard={}  inherit_from_input=off  hdl_port=on  dbl_ovrd=off  block_type=gatewayin
  adc_zcu111_m32_axis_tready : xbsIndex_r4/Gateway Out  inherit_from_input=on  hdl_port=on  rows=1  columns=1  UseAsDAC=off  DACChannel='1'  interface=None  automatic_assignment=on  address_offset=hex2dec('00')  intf_name=''  intf_description=''  timing_constraint=None  locs_specified=off  LOCs={}  io_standard={}  block_type=gatewayout
  adc_zcu111_m32_axis_tvalid : xbsIndex_r4/Gateway In  gui_display_data_type=Boolean  arith_type=Boolean  n_bits=128  bin_pt=126  preci_type=Double  exp_width=8  frac_width=24  rows=1  columns=1  quantization="Round  (unbiased: +/- Inf)"  overflow=Saturate  period=1  UseAsADC=off  ADCChannel='1'  interface=None  automatic_assignment=on  address_offset=hex2dec('00')  intf_name=''  intf_description=''  default_value=0  timing_constraint=None  locs_specified=off  LOCs={}  io_standard={}  inherit_from_input=off  hdl_port=on  dbl_ovrd=off  block_type=gatewayin
  adc_zcu111_m33_axis_tdata : xbsIndex_r4/Gateway In  gui_display_data_type=Fixed-point  arith_type="Signed  (2's comp)"  n_bits=128  bin_pt=126  preci_type=Double  exp_width=8  frac_width=24  rows=1  columns=1  quantization="Round  (unbiased: +/- Inf)"  overflow=Saturate  period=1  UseAsADC=off  ADCChannel='1'  interface=None  automatic_assignment=on  address_offset=hex2dec('00')  intf_name=''  intf_description=''  default_value=0  timing_constraint=None  locs_specified=off  LOCs={}  io_standard={}  inherit_from_input=off  hdl_port=on  dbl_ovrd=off  block_type=gatewayin
  adc_zcu111_m33_axis_tready : xbsIndex_r4/Gateway Out  inherit_from_input=on  hdl_port=on  rows=1  columns=1  UseAsDAC=off  DACChannel='1'  interface=None  automatic_assignment=on  address_offset=hex2dec('00')  intf_name=''  intf_description=''  timing_constraint=None  locs_specified=off  LOCs={}  io_standard={}  block_type=gatewayout
  adc_zcu111_m33_axis_tvalid : xbsIndex_r4/Gateway In  gui_display_data_type=Boolean  arith_type=Boolean  n_bits=128  bin_pt=126  preci_type=Double  exp_width=8  frac_width=24  rows=1  columns=1  quantization="Round  (unbiased: +/- Inf)"  overflow=Saturate  period=1  UseAsADC=off  ADCChannel='1'  interface=None  automatic_assignment=on  address_offset=hex2dec('00')  intf_name=''  intf_description=''  default_value=0  timing_constraint=None  locs_specified=off  LOCs={}  io_standard={}  inherit_from_input=off  hdl_port=on  dbl_ovrd=off  block_type=gatewayin
  m00_axis_tdata : Outport
  m00_axis_tvalid : Outport  Port=2
  m01_axis_tdata : Outport  Port=3
  m01_axis_tvalid : Outport  Port=4
  m02_axis_tdata : Outport  Port=5
  m02_axis_tvalid : Outport  Port=6
  m03_axis_tdata : Outport  Port=7
  m03_axis_tvalid : Outport  Port=8
  m10_axis_tdata : Outport  Port=9
  m10_axis_tvalid : Outport  Port=10
  m11_axis_tdata : Outport  Port=11
  m11_axis_tvalid : Outport  Port=12
  m12_axis_tdata : Outport  Port=13
  m12_axis_tvalid : Outport  Port=14
  m13_axis_tdata : Outport  Port=15
  m13_axis_tvalid : Outport  Port=16
  m20_axis_tdata : Outport  Port=17
  m20_axis_tvalid : Outport  Port=18
  m21_axis_tdata : Outport  Port=19
  m21_axis_tvalid : Outport  Port=20
  m22_axis_tdata : Outport  Port=21
  m22_axis_tvalid : Outport  Port=22
  m23_axis_tdata : Outport  Port=23
  m23_axis_tvalid : Outport  Port=24
  m30_axis_tdata : Outport  Port=25
  m30_axis_tvalid : Outport  Port=26
  m31_axis_tdata : Outport  Port=27
  m31_axis_tvalid : Outport  Port=28
  m32_axis_tdata : Outport  Port=29
  m32_axis_tvalid : Outport  Port=30
  m33_axis_tdata : Outport  Port=31
  m33_axis_tvalid : Outport  Port=32
  wires:
  adc_zcu111_m00_axis_tdata/1 -> m00_axis_tdata/1
  adc_zcu111_m01_axis_tdata/1 -> m01_axis_tdata/1
  adc_zcu111_m02_axis_tdata/1 -> m02_axis_tdata/1
  adc_zcu111_m03_axis_tdata/1 -> m03_axis_tdata/1
  adc_zcu111_m12_axis_tdata/1 -> m12_axis_tdata/1
  adc_zcu111_m13_axis_tdata/1 -> m13_axis_tdata/1
  adc_zcu111_m10_axis_tdata/1 -> m10_axis_tdata/1
  adc_zcu111_m11_axis_tdata/1 -> m11_axis_tdata/1
  adc_zcu111_m21_axis_tdata/1 -> m21_axis_tdata/1
  adc_zcu111_m22_axis_tdata/1 -> m22_axis_tdata/1
  adc_zcu111_m31_axis_tdata/1 -> m31_axis_tdata/1
  adc_zcu111_m20_axis_tdata/1 -> m20_axis_tdata/1
  adc_zcu111_m33_axis_tdata/1 -> m33_axis_tdata/1
  adc_zcu111_m23_axis_tdata/1 -> m23_axis_tdata/1
  adc_zcu111_m30_axis_tdata/1 -> m30_axis_tdata/1
  adc_zcu111_m32_axis_tdata/1 -> m32_axis_tdata/1
  adc_zcu111_m21_axis_tvalid/1 -> m21_axis_tvalid/1
  adc_zcu111_m12_axis_tvalid/1 -> m12_axis_tvalid/1
  adc_zcu111_m03_axis_tvalid/1 -> m03_axis_tvalid/1
  adc_zcu111_m20_axis_tvalid/1 -> m20_axis_tvalid/1
  adc_zcu111_m30_axis_tvalid/1 -> m30_axis_tvalid/1
  adc_zcu111_m10_axis_tvalid/1 -> m10_axis_tvalid/1
  adc_zcu111_m13_axis_tvalid/1 -> m13_axis_tvalid/1
  adc_zcu111_m00_axis_tvalid/1 -> m00_axis_tvalid/1
  adc_zcu111_m11_axis_tvalid/1 -> m11_axis_tvalid/1
  adc_zcu111_m02_axis_tvalid/1 -> m02_axis_tvalid/1
  adc_zcu111_m01_axis_tvalid/1 -> m01_axis_tvalid/1
  adc_zcu111_m22_axis_tvalid/1 -> m22_axis_tvalid/1
  adc_zcu111_m31_axis_tvalid/1 -> m31_axis_tvalid/1
  adc_zcu111_m33_axis_tvalid/1 -> m33_axis_tvalid/1
  adc_zcu111_m23_axis_tvalid/1 -> m23_axis_tvalid/1
  adc_zcu111_m32_axis_tvalid/1 -> m32_axis_tvalid/1
  m00_axis_tready/1 -> adc_zcu111_m00_axis_tready/1
  m01_axis_tready/1 -> adc_zcu111_m01_axis_tready/1
  m02_axis_tready/1 -> adc_zcu111_m02_axis_tready/1
  m03_axis_tready/1 -> adc_zcu111_m03_axis_tready/1
  m12_axis_tready/1 -> adc_zcu111_m12_axis_tready/1
  m11_axis_tready/1 -> adc_zcu111_m11_axis_tready/1
  m10_axis_tready/1 -> adc_zcu111_m10_axis_tready/1
  m13_axis_tready/1 -> adc_zcu111_m13_axis_tready/1
  m33_axis_tready/1 -> adc_zcu111_m33_axis_tready/1
  m30_axis_tready/1 -> adc_zcu111_m30_axis_tready/1
  m32_axis_tready/1 -> adc_zcu111_m32_axis_tready/1
  m22_axis_tready/1 -> adc_zcu111_m22_axis_tready/1
  m20_axis_tready/1 -> adc_zcu111_m20_axis_tready/1
  m31_axis_tready/1 -> adc_zcu111_m31_axis_tready/1
  m23_axis_tready/1 -> adc_zcu111_m23_axis_tready/1
  m21_axis_tready/1 -> adc_zcu111_m21_axis_tready/1
